simulink model "BB_control_SIM_A_x (1)"  (R2024b)
settings: Solver=ode4  StartTime=0.0  StopTime=20  FixedStep=1e-5  RelTol=1e-3
undefined symbols (not defined in the file or in its folder): iL0, tref, vo0, vref
settings Model: Creator=gerardo.flores  LastModifiedBy=gerardo.flores

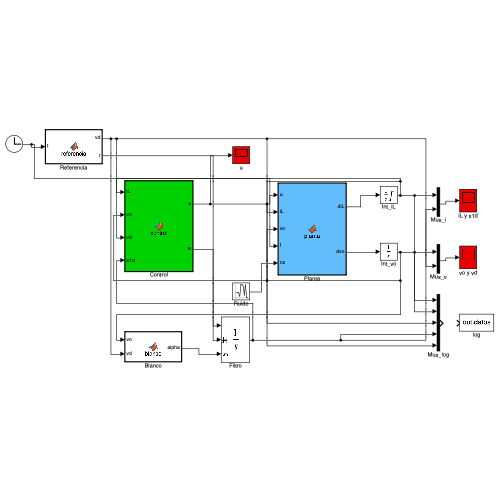
[thumbnail: Simulink's stored preview of the top-level diagram]
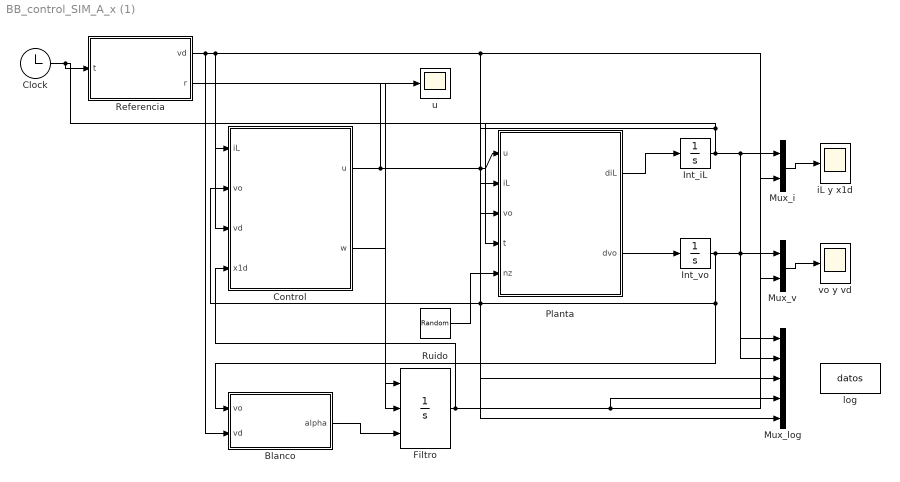
== system BB_control_SIM_A_x (1) ==
  Blanco : MATLAB Function  TreatAsAtomicUnit=on
  Clock : Clock
  Control : MATLAB Function  TreatAsAtomicUnit=on
  Filtro : Integrator  ExternalReset=either  InitialConditionSource=external
  Int_iL : Integrator  InitialCondition=iL0  LimitOutput=on  LowerSaturationLimit=0
  Int_vo : Integrator  InitialCondition=vo0
  Mux_i : Mux  Inputs=2
  Mux_log : Mux  Inputs=5
  Mux_v : Mux  Inputs=2
  Planta : MATLAB Function  TreatAsAtomicUnit=on
  Referencia : MATLAB Function  TreatAsAtomicUnit=on
  Ruido : RandomNumber  Variance=0.01  Seed=7  SampleTime=1e-4
  iL y x1d : Scope
  log : ToWorkspace  VariableName=datos  SaveFormat=Structure With Time  SampleTime=-1
      settings: Decimation=10
  u : Scope
  vo y vd : Scope
  wires:
  Clock/1 -> Referencia/1(t), Planta/4(t)
  Referencia/1(vd) -> Mux_v/2, Mux_log/3, Control/3(vd), Blanco/2(vd)
  Referencia/2(r) -> Filtro/2
  Blanco/1(alpha) -> Filtro/3
  Control/2(w) -> Filtro/1
  Filtro/1 -> Mux_i/2, Mux_log/4, Control/4(x1d)
  Control/1(u) -> Planta/1(u), Mux_log/5, u/1
  Ruido/1 -> Planta/5(nz)
  Planta/1(diL) -> Int_iL/1
  Planta/2(dvo) -> Int_vo/1
  Int_iL/1 -> Mux_i/1, Mux_log/1, Control/1(iL), Planta/2(iL)
  Int_vo/1 -> Control/2(vo), Planta/3(vo), Blanco/1(vo), Mux_v/1, Mux_log/2
  Mux_v/1 -> vo y vd/1
  Mux_i/1 -> iL y x1d/1

== matlab function BB_control_SIM_A_x (1)/Blanco ==
  data: vo input; alpha output; vd input; P parameter
function alpha = blanco(vo, vd, P)
% Blanco virtual (condicion inicial y reinicio del filtro)
En=P(1); Cn=P(3); Rn=P(4); k2=P(6); ep=P(7);
q  = 1 - vd/(vd - En);
e2 = vo - vd;
alpha = (Cn/q)*(k2*e2/(e2^2 + ep^2)^(1/4) - vo/(Rn*Cn));
end

== matlab function BB_control_SIM_A_x (1)/Referencia ==
  data: t input; vd output; r output; tref parameter; vref parameter
function [vd, r] = referencia(t, tref, vref)
% Referencia por tramos; r cambia 0/1 en cada escalon (reinicia el filtro)
k = 1;
for i = 2:numel(tref)
    if t >= tref(i)
        k = i;
    end
end
vd = vref(k);
r  = mod(k, 2);
end

== matlab function BB_control_SIM_A_x (1)/Control ==
  data: iL input; u output; vo input; vd input; x1d input; w output; P parameter
function [u, w] = control(iL, vo, vd, x1d, P)
% Control para el buck-boost inversor. P = [En Ln Cn Rn k1 k2 eps tau ell M]
En=P(1); Ln=P(2); Cn=P(3); Rn=P(4); 

k1=P(5); k2=P(6); ep=P(7); 
tau=P(8); ell=P(9); M=P(10);

q  = 1 - vd/(vd - En);                         % 1 - u* (constante)
e2 = vo - vd;
K  = k2*e2/(e2^2 + ep^2)^(1/4);
alpha = (Cn/q)*(K - vo/(Rn*Cn));               % blanco virtual
w  = (alpha - x1d)/tau;                        % entrada del filtro = derivada de x1d
e1 = iL - x1d;
s  = 1 + (Ln*k1*sign(e1)*sqrt(abs(e1)) + En - Ln*w)/(vo - En);
cs = pi/(2*(M - ell));                         % saturacion de dos lados
if s <= 0
    u = 0;
elseif s < ell
    u = s;
else
    u = ell + tanh(cs*(s - ell))/cs;
end
end

== matlab function BB_control_SIM_A_x (1)/Planta ==
  data: u input; diL output; iL input; vo input; t input; nz input; dvo output; Pp parameter
function [diL, dvo] = planta(u, iL, vo, t, nz, Pp)
% Modelo promediado del buck-boost inversor (vo < 0) con los perfiles de la Fig. 4
E=Pp(1); L=Pp(2); C=Pp(3); R=Pp(4); perfil=Pp(5); D=0;
if perfil >= 1                                 % Escenarios A y B
    E = 12 + 0.3*sin(2*pi*t/20);
    D = 1.75*sin(2*pi*t/4.2) - 0.25;
    if t >= 5 && t < 5.2
        D = D + 10.5*(t - 5)/0.2;
    end
end
if perfil >= 2                                 % solo Escenario A
    R = 25 + 3*sin(2*pi*t/4.2);
    L = 5e-3 + 0.5e-3*sin(2*pi*t/12.6);
    if t < 9
        C = 950e-6;
    else
        C = 500e-6;
    end
end
diL = ((1-u)*vo + u*E)/L;
if iL <= 0 && diL < 0
    diL = 0;                                   % diodo: iL no se hace negativa
end
dvo = -(1-u)*iL/C - vo/(R*C) + D + (perfil >= 1)*nz;
end
